simulink model "modele_moteur"  (R2026b)
settings: Solver=VariableStepAuto
undefined symbols (not defined in the file or in its folder): pwm_pct
settings Model: Creator=yessi  LastModifiedBy=yessi

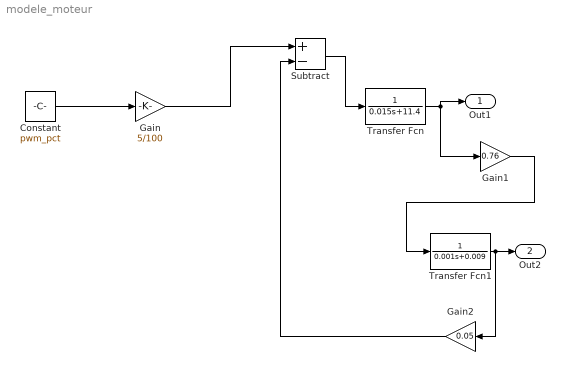
== system modele_moteur ==
  Constant : Constant  Value=pwm_pct  VectorParams1D=off
  Gain : Gain  Gain=5/100
  Gain1 : Gain  Gain=0.76
  Gain2 : Gain  Gain=0.05
  Subtract : Sum  Inputs=+-
  Transfer Fcn : TransferFcn  Denominator=[0.015 11.4]
  Transfer Fcn1 : TransferFcn  Denominator=[0.001 0.009]
  Out1 : Outport
  Out2 : Outport  Port=2
  wires:
  Constant/1 -> Gain/1
  Gain/1 -> Subtract/1
  Subtract/1 -> Transfer Fcn/1
  Transfer Fcn/1 -> Gain1/1, Out1/1
  Gain1/1 -> Transfer Fcn1/1
  Transfer Fcn1/1 -> Gain2/1, Out2/1
  Gain2/1 -> Subtract/2
